simulink model "sschdlexPMSMDriveOptimizedMotor"  (R2026a)
settings: Solver=FixedStepDiscrete  StopTime=0.6  AbsTol=1e-3
PreLoadFcn:
  | % Control parameters
  | Ts = 1e-6;   % Fundamental sample time
  | fsw = 25e3;   % Switching frequency (Hz)
  | fc = fsw*10; % Control loop frequency (Hz)
  | Tsc = 1/fc;  % Control loop sample time
  | 
  | % PMSM parameters
  | PM = 0.03; % Permanent magnet flux linkage
  | Ld = 2e-4;  % d-axis inductance
  | Lq = 2e-4;  % q-axis inductance
  | L0 = 2e-4;  % 0-axis inductance
  | Rs = 0.013; % Stator resistance
  | N = 6; % Number of pole pairs
  | J = 0.2; % Moment of inertia
  | 
  | % Operating and derived limits
  | Imax = 100;  % Max stator current (peak value)
  | Tmax = 1.5*N*PM*Imax; % Max lectromagnetic torque
  | fnom = 100;  % Nominal frequency (Hz)
  | rpm_nom = 60*fnom/N;      % Nominal rotor speed (rpm)
  | omegam_nom = 2*pi*fnom/N; % Nominal mechanical rotor speed
  | Pmax = omegam_nom*Tmax;     % Maximum power
  | 
  | Gs = 4.4526;
  | s = 2.8994;
  | h = 2e-6;
PostLoadFcn:
  | SimscapePlant_SolverConfiguration_Gs = Simulink.Parameter;
  | SimscapePlant_SolverConfiguration_Gs.Value = 1;
  | SimscapePlant_SolverConfiguration_Gs.CoderInfo.StorageClass = 'ExportedGlobal';
  | SimscapePlant_SolverConfiguration_s = Simulink.Parameter;
  | SimscapePlant_SolverConfiguration_s.Value = 1;
  | SimscapePlant_SolverConfiguration_s.CoderInfo.StorageClass = 'ExportedGlobal';SimscapePlant_PermanentMagnetSynchronousMotor_NPP = Simulink.Parameter;
  | SimscapePlant_PermanentMagnetSynchronousMotor_NPP.Value = 6;
  | SimscapePlant_PermanentMagnetSynchronousMotor_NPP.CoderInfo.StorageClass = 'ExportedGlobal';SimscapePlant_PermanentMagnetSynchronousMotor_Lambda_pm = Simulink.Parameter;
  | SimscapePlant_PermanentMagnetSynchronousMotor_Lambda_pm.Value = 0.03;
  | SimscapePlant_PermanentMagnetSynchronousMotor_Lambda_pm.CoderInfo.StorageClass = 'ExportedGlobal';SimscapePlant_PermanentMagnetSynchronousMotor_Ld = Simulink.Parameter;
  | SimscapePlant_PermanentMagnetSynchronousMotor_Ld.Value = 0.0002;
  | SimscapePlant_PermanentMagnetSynchronousMotor_Ld.CoderInfo.StorageClass = 'ExportedGlobal';SimscapePlant_PermanentMagnetSynchronousMotor_Lq = Simulink.Parameter;
  | SimscapePlant_PermanentMagnetSynchronousMotor_Lq.Value = 0.0002;
  | SimscapePlant_PermanentMagnetSynchronousMotor_Lq.CoderInfo.StorageClass = 'ExportedGlobal';SimscapePlant_PermanentMagnetSynchronousMotor_Rs = Simulink.Parameter;
  | SimscapePlant_PermanentMagnetSynchronousMotor_Rs.Value = 0.013;
  | SimscapePlant_PermanentMagnetSynchronousMotor_Rs.CoderInfo.StorageClass = 'ExportedGlobal';
libraries: SimscapeFPGAHIL_lib x13, nesl_utility x7, fl_lib x6, ee_lib x3, eePmsmFieldOrientedControl x1, batteryecm_lib x1
Description:
  | Three-Phase PMSM Drive
settings Model: DataTypeOverride=Off  Creator=The MathWorks, Inc.  LastModifiedBy=The MathWorks, Inc.
settings SolverCC: MaxConsecutiveMinStep=2  ZeroCrossAlgorithm=Adaptive
settings DataIOCC: MaxDataPoints=690000  SignalLoggingName=logsout_ee_pmsm_drive
settings OptimizationCC: ConditionallyExecuteInputs=off  InheritOutputTypeSmallerThanSingle=on
settings DebuggingCC: AlgebraicLoopMsg=error  MaxConsecutiveZCsMsg=none  IgnoredZcDiagnostic=none  SingleTaskRateTransMsg=error  ParameterPrecisionLossMsg=none  PregeneratedLibrarySubsystemCodeDiagnostic=none
settings HardwareCC: ProdHWDeviceType=ASIC/FPGA->ASIC/FPGA  TargetBitPerLong=64.0  TargetBitPerPointer=64.0  TargetBitPerSizeT=64.0  TargetBitPerPtrDiffT=64.0  TargetLongLongMode=on  TargetIntDivRoundTo=Zero  TargetEndianess=LittleEndian  TargetWordSize=64.0  TargetHWDeviceType=Custom Processor->MATLAB Host Computer  ProdEqTarget=off
settings SimscapeCC: SimscapeNominalValues="[{\"value\":\"1\",\"unit\":\"A\"},{\"value\":\"1\",\"unit\":\"bar\"},{\"value\":\"1\",\"unit\":\"cm^2\"},{\"value\":\"1\",\"unit\":\"cm^3/s\"},{\"value\":\"1\",\"unit\":\"kJ/kg\"},{\"value\":\"1\",\"unit\":\"kW\"},{\"value\":\"1\",\"unit\":\"l\"},{\"value\":\"1\",\"unit\":\"N\"},{\"value\":\"1\",\"unit\":\"N*m\"},{\"value\":\"1\",\"unit\":\"V\"}]"  SimscapeLogSimulationStatistics=on  SimscapeLogName=simlog_ee_pmsm_drive  SimscapeLogDataHistory=690000.0

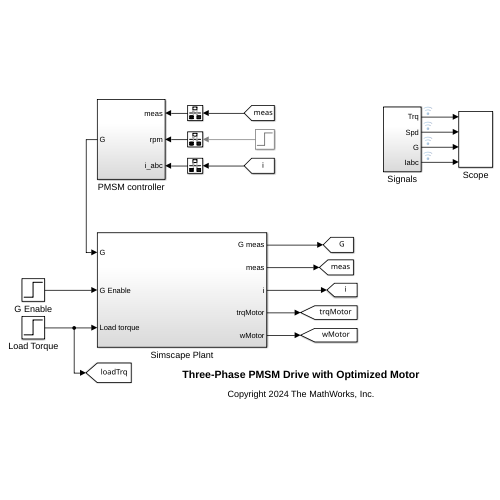
[thumbnail: Simulink's stored preview of the top-level diagram]
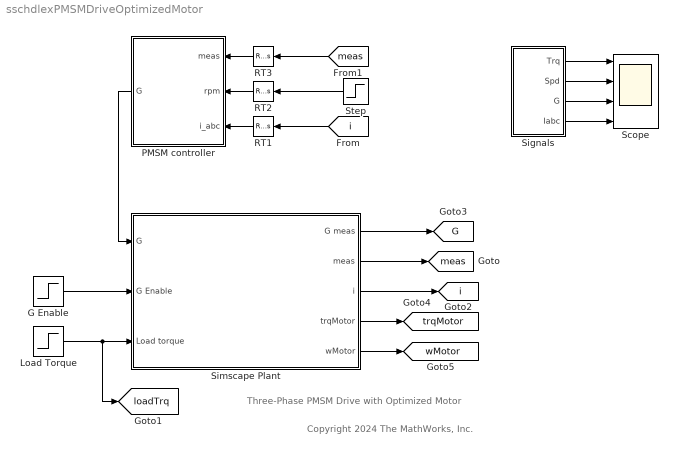
== system sschdlexPMSMDriveOptimizedMotor ==
  note: Three-Phase PMSM Drive with Optimized Motor
  note: Copyright 2024 The MathWorks, Inc.
  G Enable : Step  Time=1e-4  SampleTime=Ts
  Load Torque : Step  Time=0.1  FinalValue=5  SampleTime=Ts
  PMSM controller : Subsystem
  RT1 : RateTransition  OutPortSampleTime=Tsc
  RT2 : RateTransition  OutPortSampleTime=Tsc
  RT3 : RateTransition  OutPortSampleTime=Tsc
  Scope : Scope  NumInputPorts=4
      settings: Title=Demanded and achieved torques  ActiveDisplayYMinimum=-0.625  ActiveDisplayYMaximum=5.625
  "Signals " : Subsystem
  Simscape Plant : Subsystem
  Step : Step  Time=0.1  FinalValue=500  SampleTime=0
  tag scope: G=global, i=global, loadTrq=global, meas=global, trqMotor=global, wMotor=global
  wires:
  Step/1 -> RT2/1
  RT3/1 -> PMSM controller/1(meas)
  RT2/1 -> PMSM controller/2(rpm)
  RT1/1 -> PMSM controller/3(i_abc)
  "Signals "/2(Spd) -> Scope/2
  "Signals "/4(Iabc) -> Scope/4
  "Signals "/3(G) -> Scope/3
  "Signals "/1(Trq) -> Scope/1
  [i] -> RT1/1
  [meas] -> RT3/1
  PMSM controller/1(G) -> Simscape Plant/1(G)
  G Enable/1 -> Simscape Plant/2(G Enable)
  Load Torque/1 -> [loadTrq], Simscape Plant/3(Load torque)
  Simscape Plant/2(meas) -> [meas]
  Simscape Plant/3(i) -> [i]
  Simscape Plant/1(G meas) -> [G]
  Simscape Plant/4(trqMotor) -> [trqMotor]
  Simscape Plant/5(wMotor) -> [wMotor]

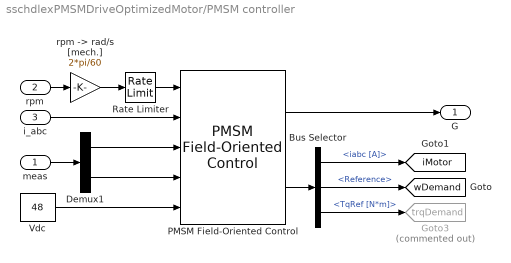
== system sschdlexPMSMDriveOptimizedMotor/PMSM controller ==
  meas : Inport
  rpm : Inport  Port=2
  i_abc : Inport  Port=3
  Bus Selector : BusSelector  OutputSignals=iabc [A],Reference,TqRef [N*m]
  Demux1 : Demux  Outputs=2
  Goto3 : Goto  Commented=on  GotoTag=trqDemand  TagVisibility=global
  PMSM Field-Oriented Control : eePmsmFieldOrientedControl/PMSM Field-Oriented Control  winding_type=Wye-wound  CtrlMode=Velocity control  Vnom=48  Pmax=Pmax  Tmax=Tmax*1.5  p=N  Vdc_on=10  Ts=Ts  Tsc=Tsc  CtrlType=PI control  Kp_w=60  Ki_w=300*2  Kv_w=1  Kaw_w=1000  RefType=Zero d-axis control  rpmVec=[0, 3000]  TqVec=[-100, 0, 100]  VdcVec=[300, 350]  PWMMode=SPWM: sinusoidal PWM  ModFactor=1  idMatrix=zeros(2,3,2)  iqMatrix=zeros(2,3,2)  psim=PM  Ld=0.00024  Lq=0.00029  Rs=0.01  AxisAlignment=Q-axis  Kp_id=0.1  Ki_id=10  Kaw_id=1000  Kp_iq=0.1  Ki_iq=10  Kaw_iq=1000  AxisPrio=Q-axis  ActZC=off  ActFF=on  ParamTypeFF=Constant parameters  LdFF=Ld  LqFF=Lq  psimFF=PM  idVect=[-200, 0, 200]  iqVect=[-200, 0, 200]  LdMatrix=0.0002 * ones(3, 3)  LqMatrix=0.0002 * ones(3, 3)  psimMatrix=0.04 * ones(3, 3)  CPWMMode=SPWM: sinusoidal PWM  fsw=fsw
  Rate Limiter : RateLimiter  RisingSlewLimit=Tmax/J  FallingSlewLimit=-Tmax/J  SampleTimeMode=inherited
  Vdc : Constant  Value=48  SampleTime=Tsc
  "rpm -> rad/s [mech.]" : Gain  Gain=2*pi/60
  G : Outport  VectorParamsAs1DForOutWhenUnconnected=off
  tag scope: iMotor=global, wDemand=global
  wires:
  PMSM Field-Oriented Control/1 -> G/1
  Vdc/1 -> PMSM Field-Oriented Control/5
  PMSM Field-Oriented Control/2 -> Bus Selector/1
  i_abc/1 -> PMSM Field-Oriented Control/2
  meas/1 -> Demux1/1
  Demux1/1 -> PMSM Field-Oriented Control/3
  Demux1/2 -> PMSM Field-Oriented Control/4
  Bus Selector/1 -> [iMotor]  "<iabc [A]>"
  Bus Selector/2 -> [wDemand]  "<Reference>"
  Bus Selector/3 -> Goto3/1  "<TqRef [N*m]>"
  rpm/1 -> "rpm -> rad/s [mech.]"/1
  Rate Limiter/1 -> PMSM Field-Oriented Control/1
  "rpm -> rad/s [mech.]"/1 -> Rate Limiter/1

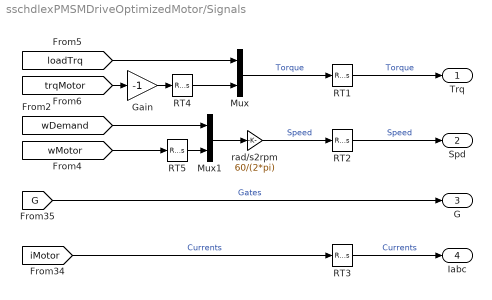
== system sschdlexPMSMDriveOptimizedMotor/Signals  ==
  Gain : Gain  Gain=-1
  Mux : Mux  Inputs=2
  Mux1 : Mux  Inputs=2
  RT{1..4} (4 alike) : RateTransition  OutPortSampleTime=Ts
  RT5 : RateTransition  OutPortSampleTime=Tsc
  rad/s2rpm : Gain  Gain=60/(2*pi)
  Trq : Outport  VectorParamsAs1DForOutWhenUnconnected=off
  Spd : Outport  Port=2  VectorParamsAs1DForOutWhenUnconnected=off
  G : Outport  Port=3  VectorParamsAs1DForOutWhenUnconnected=off
  Iabc : Outport  Port=4  VectorParamsAs1DForOutWhenUnconnected=off
  wires:
  [loadTrq] -> Mux/1
  [G] -> G/1  "Gates"
  Mux1/1 -> rad/s2rpm/1
  Mux/1 -> RT1/1  "Torque"
  [iMotor] -> RT3/1  "Currents"
  [wDemand] -> Mux1/1
  rad/s2rpm/1 -> RT2/1  "Speed"
  [trqMotor] -> Gain/1
  [wMotor] -> RT5/1
  RT1/1 -> Trq/1  "Torque"
  RT2/1 -> Spd/1  "Speed"
  RT3/1 -> Iabc/1  "Currents"
  RT4/1 -> Mux/2
  RT5/1 -> Mux1/2
  Gain/1 -> RT4/1

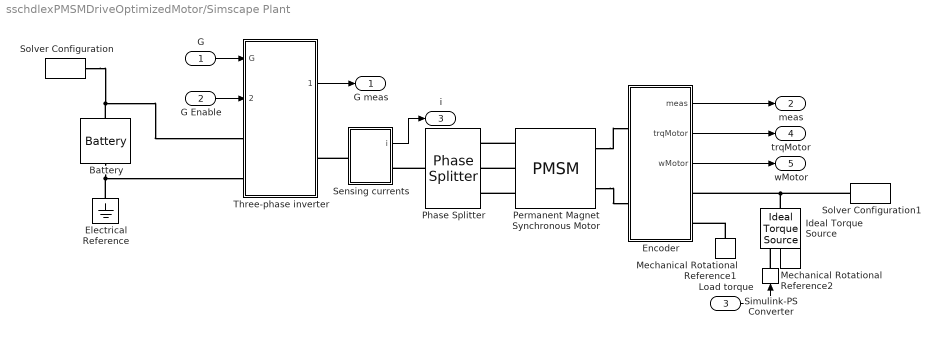
== system sschdlexPMSMDriveOptimizedMotor/Simscape Plant ==
  G : Inport
  G Enable : Inport  Port=2
  Load torque : Inport  Port=3
  Battery : batteryecm_lib/Battery  Vnom=48 V  prm_dir=1  R1_dis=2 Ohm  R1_ch=2 Ohm  R1=0.001 Ohm  prm_AH=1  AH=14000 hr*A  V1=470 V  AH1=5000 hr*A  prm_R2=1  R2=inf Ohm  Tmeas=298.15 K  charge_measurement_port=simscape.enum.battery.enable.no  prm_dyn=1  Rp1=0.005 Ohm  tau1=30 s  Rp2=0.005 Ohm  tau2=30 s  Rp3=0.005 Ohm  tau3=30 s  Rp4=0.005 Ohm  tau4=30 s  Rp5=0.005 Ohm  tau5=30 s  prm_fade=1  N_fade=100  AH_fade=45 hr*A  R1_fade=2.02 Ohm  R1_ch_fade=2.02 Ohm  V1_fade=10.35 V  prm_age=1  prm_age_OCV=1  OCV_age=0.9  SOC_age=60  Tmeas_age=298.15 K  delta_time_age_vec=[0] d  temperature_age_vec=[273] K  OCV_scaling_age=2.2134e6  OCV_offset_age=1.632e6  temp_exp_age=0.515833569 V  t_exp_age=0.75  Vnom_T2=12 V  R1_T2=2.2 Ohm  R1_T2_dis=2.2 Ohm  R1_T2_ch=2.2 Ohm  V1_T2=11.4 V  R2_T2=2200 Ohm  Rp1_T2=0.005 Ohm  tau1_T2=30 s  Rp2_T2=0.005 Ohm  tau2_T2=30 s  Rp3_T2=0.005 Ohm  tau3_T2=30 s  Rp4_T2=0.005 Ohm  tau4_T2=30 s  Rp5_T2=0.005 Ohm  tau5_T2=30 s  Tmeas2=273.15 K  thermal_port=simscape.enum.thermaleffects.omit  thermal_mass=30000 J/K  i_specify=off  i_priority=None  i=0 A  i_nominal_specify=off  i_nominal_value=1  i_nominal_unit=A  v_specify=off  v_priority=None  v=0 V  v_nominal_specify=off  v_nominal_value=1  v_nominal_unit=V  charge_specify=on  charge_priority=High  charge=7000 hr*A  charge_nominal_specify=off  charge_nominal_value=1  charge_nominal_unit=A*hr  num_cycles_specify=off  num_cycles_priority=High  num_cycles=0  num_cycles_nominal_specify=off  num_cycles_nominal_value=1  num_cycles_nominal_unit=1  temperature_specify=off  temperature_priority=High  temperature=298.15 K  temperature_nominal_specify=off  temperature_nominal_value=1  temperature_nominal_unit=K
  Electrical Reference : fl_lib/Electrical/Electrical Elements/Electrical Reference
  Encoder : Subsystem
  Ideal Torque Source : fl_lib/Mechanical/Mechanical Sources/Ideal Torque Source
  Mechanical Rotational Reference1 : fl_lib/Mechanical/Rotational Elements/Mechanical Rotational Reference
  Mechanical Rotational Reference2 : fl_lib/Mechanical/Rotational Elements/Mechanical Rotational Reference
  Permanent Magnet Synchronous Motor : SimscapeFPGAHIL_lib/PMSM Motor/PMSM  NPP=SimscapePlant_PermanentMagnetSynchronousMotor_NPP  Lambda_pm=SimscapePlant_PermanentMagnetSynchronousMotor_Lambda_pm  Ld=SimscapePlant_PermanentMagnetSynchronousMotor_Ld  Lq=SimscapePlant_PermanentMagnetSynchronousMotor_Lq  Rs=SimscapePlant_PermanentMagnetSynchronousMotor_Rs  J=0.2  winding=Wye  Load_type=Torque-driven  Ts=Ts  torque_initial=0  i_d_initial=0  i_q_initial=0  angular_position_initial=0  angular_velocity_initial=0
  Phase Splitter : ee_lib/Connectors & References/Phase Splitter
  Sensing currents : Subsystem
      mask Display: disp('i')
  Simulink-PS Converter : nesl_utility/Simulink-PS Converter  PhysicalDomain=network_engine_domain  SubClassName=ps_input  LeftPortType=input  RightPortType=output  PseudoPeriodic=off  Frequencies=[]  NoiseDistribution=none  NoiseParameters=[]  Unit=1  AffineConversion=off  FilteringAndDerivatives=provide  SimscapeFilterOrder=1  InputFilterTimeConstant=0.001  UdotUserProvided=0
  Solver Configuration : nesl_utility/Solver Configuration  PhysicalDomain=network_engine_domain  SubClassName=solver  LeftPortType=input  RightPortType=generic  Tones=[]  Harmonics=[]  SimulateNoise=off  Profile=off  UseLocalSampling=off  EnableSwitchedLinearOptims=on  FrequencyDomain=off  UseCCode=off  RelTol=0.001  AbsTol=1e-06  MinStep=1e-09  ToWorkspace=off  RevertToSquareIcSolve=off  NumHomotopyIterations=100  PhasorMode=off  PhasorModeNumHarmonics=1  ConsistencySolver=NEWTON_FTOL  CanonicalOrdering=UNORDERED  OptimizeIntermediates=UNOPTIMIZED  IndexReductionMethod=DerivativeReplacement  DoDC=off  ResidualTolerance=1e-9  ConsistencyTolSource=GLOBAL  ConsistencyAbsTol=0.001  ConsistencyRelTol=0.001  ConsistencyTolFactor=0.001  UseLocalSolver=on  LocalSolverChoice=NE_BACKWARD_EULER_ADVANCER  ResolveIndetEquations=on  FunctionEvalNumThread=1  LocalSolverSampleTime=Ts  DoFixedCost=on  MaxNonlinIter=4  MaxModeIter=2  ComputeImpulses=off  ImpulseIterations=2  LinearAlgebra=auto  LinearAlgebraNumThread=0  EquationFormulation=NE_TIME_EF  DelaysMemoryBudget=1024  AutomaticFiltering=on  FilteringTimeConstant=0.001  PartitionStorageMethod=AS_NEEDED  PartitionMemoryBudget=1024  PartitionMethod=FAST  MultibodyUseLocalSolver=off  MultibodyLocalSolverChoice=ODE1  MultibodyLocalSolverSampleTime=0.001
  Solver Configuration1 : nesl_utility/Solver Configuration  PhysicalDomain=network_engine_domain  SubClassName=solver  LeftPortType=input  RightPortType=generic  Tones=[]  Harmonics=[]  SimulateNoise=off  Profile=off  UseLocalSampling=off  EnableSwitchedLinearOptims=on  FrequencyDomain=off  UseCCode=off  RelTol=0.001  AbsTol=1e-06  MinStep=1e-09  ToWorkspace=off  RevertToSquareIcSolve=off  NumHomotopyIterations=100  PhasorMode=off  PhasorModeNumHarmonics=1  ConsistencySolver=NEWTON_FTOL  CanonicalOrdering=UNORDERED  OptimizeIntermediates=UNOPTIMIZED  IndexReductionMethod=DerivativeReplacement  DoDC=off  ResidualTolerance=1e-9  ConsistencyTolSource=GLOBAL  ConsistencyAbsTol=0.001  ConsistencyRelTol=0.001  ConsistencyTolFactor=0.001  UseLocalSolver=on  LocalSolverChoice=NE_BACKWARD_EULER_ADVANCER  ResolveIndetEquations=on  FunctionEvalNumThread=1  LocalSolverSampleTime=Ts  DoFixedCost=on  MaxNonlinIter=4  MaxModeIter=2  ComputeImpulses=off  ImpulseIterations=2  LinearAlgebra=auto  LinearAlgebraNumThread=0  EquationFormulation=NE_TIME_EF  DelaysMemoryBudget=1024  AutomaticFiltering=on  FilteringTimeConstant=0.001  PartitionStorageMethod=AS_NEEDED  PartitionMemoryBudget=1024  PartitionMethod=FAST  MultibodyUseLocalSolver=off  MultibodyLocalSolverChoice=ODE1  MultibodyLocalSolverSampleTime=0.001
  Three-phase inverter : Subsystem
  G meas : Outport
  meas : Outport  Port=2
  i : Outport  Port=3
  trqMotor : Outport  Port=4
  wMotor : Outport  Port=5
  wires:
  G Enable/1 -> Three-phase inverter/2(G Enable)
  Load torque/1 -> Simulink-PS Converter/1
  Encoder/1(meas) -> meas/1
  G/1 -> Three-phase inverter/1(G)
  Sensing currents/1(i) -> i/1
  Three-phase inverter/1(G meas) -> G meas/1
  Encoder/3(wMotor) -> wMotor/1
  Encoder/2(trqMotor) -> trqMotor/1
  connections:
  Solver Configuration/RConn1 -- Three-phase inverter/LConn1 -- Battery/LConn1
  Mechanical Rotational Reference1/LConn1 -- Encoder/RConn2
  Sensing currents/LConn1 -- Three-phase inverter/RConn1
  Ideal Torque Source/RConn2 -- Mechanical Rotational Reference2/LConn1
  Ideal Torque Source/LConn1 -- Encoder/RConn1 -- Solver Configuration1/RConn1
  Simulink-PS Converter/RConn1 -- Ideal Torque Source/RConn1
  Electrical Reference/LConn1 -- Battery/RConn1 -- Three-phase inverter/LConn2
  Phase Splitter/LConn1 -- Sensing currents/RConn1
  Permanent Magnet Synchronous Motor/RConn2 -- Encoder/LConn2
  Permanent Magnet Synchronous Motor/LConn2 -- Phase Splitter/RConn2
  Permanent Magnet Synchronous Motor/RConn1 -- Encoder/LConn1
  Permanent Magnet Synchronous Motor/LConn1 -- Phase Splitter/RConn1
  Permanent Magnet Synchronous Motor/LConn3 -- Phase Splitter/RConn3

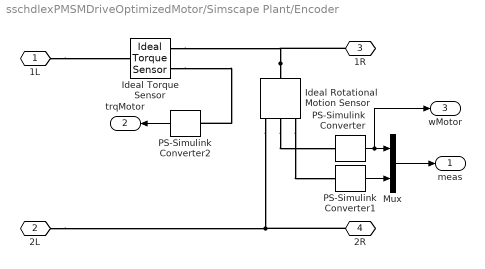
== system sschdlexPMSMDriveOptimizedMotor/Simscape Plant/Encoder ==
  Ideal Rotational Motion Sensor : fl_lib/Mechanical/Mechanical Sensors/Ideal Rotational Motion Sensor  reference=foundation.enum.MeasurementReference.difference  acceleration_port=false  velocity_port=true  position_port=true  wrap_angle=simscape.enum.onoff.off  offset=0 deg
  Ideal Torque Sensor : fl_lib/Mechanical/Mechanical Sensors/Ideal Torque Sensor
  Mux : Mux  Inputs=2
  PS-Simulink Converter : nesl_utility/PS-Simulink Converter  PhysicalDomain=network_engine_domain  SubClassName=ps_output  LeftPortType=input  RightPortType=output  PseudoPeriodic=off  Frequencies=[]  VectorFormat=1-D array  Unit=rad/s  AffineConversion=off
  PS-Simulink Converter1 : nesl_utility/PS-Simulink Converter  PhysicalDomain=network_engine_domain  SubClassName=ps_output  LeftPortType=input  RightPortType=output  PseudoPeriodic=off  Frequencies=[]  VectorFormat=1-D array  Unit=rad  AffineConversion=off
  PS-Simulink Converter2 : nesl_utility/PS-Simulink Converter  PhysicalDomain=network_engine_domain  SubClassName=ps_output  LeftPortType=input  RightPortType=output  PseudoPeriodic=off  Frequencies=[]  VectorFormat=1-D array  Unit=N*m  AffineConversion=off
  1L : PMIOPort  Side=Left
  2L : PMIOPort  Port=2  Side=Left
  1R : PMIOPort  Port=3  Side=Right
  2R : PMIOPort  Port=4  Side=Right
  meas : Outport  VectorParamsAs1DForOutWhenUnconnected=off
  trqMotor : Outport  Port=2
  wMotor : Outport  Port=3
  wires:
  PS-Simulink Converter2/1 -> trqMotor/1
  Mux/1 -> meas/1
  PS-Simulink Converter1/1 -> Mux/2
  PS-Simulink Converter/1 -> wMotor/1, Mux/1
  connections:
  Ideal Torque Sensor/RConn2 -- PS-Simulink Converter2/LConn1
  1L/RConn1 -- Ideal Torque Sensor/LConn1
  2R/RConn1 -- 2L/RConn1 -- Ideal Rotational Motion Sensor/RConn1
  Ideal Rotational Motion Sensor/LConn1 -- 1R/RConn1 -- Ideal Torque Sensor/RConn1
  Ideal Rotational Motion Sensor/RConn2 -- PS-Simulink Converter/LConn1
  Ideal Rotational Motion Sensor/RConn3 -- PS-Simulink Converter1/LConn1

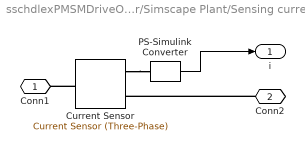
== system sschdlexPMSMDriveOptimizedMotor/Simscape Plant/Sensing currents ==
  Current Sensor : ee_lib/Sensors & Transducers/Current Sensor (Three-Phase)  port_option=ee.enum.threePhasePort.composite
  PS-Simulink Converter : nesl_utility/PS-Simulink Converter  PhysicalDomain=network_engine_domain  SubClassName=ps_output  LeftPortType=input  RightPortType=output  PseudoPeriodic=off  Frequencies=[]  VectorFormat=1-D array  Unit=A  AffineConversion=off
  Conn1 : PMIOPort  Side=Left
  Conn2 : PMIOPort  Port=2  Side=Right
  i : Outport
  wires:
  PS-Simulink Converter/1 -> i/1
  connections:
  Current Sensor/RConn1 -- PS-Simulink Converter/LConn1
  Conn2/RConn1 -- Current Sensor/RConn2
  Current Sensor/LConn1 -- Conn1/RConn1

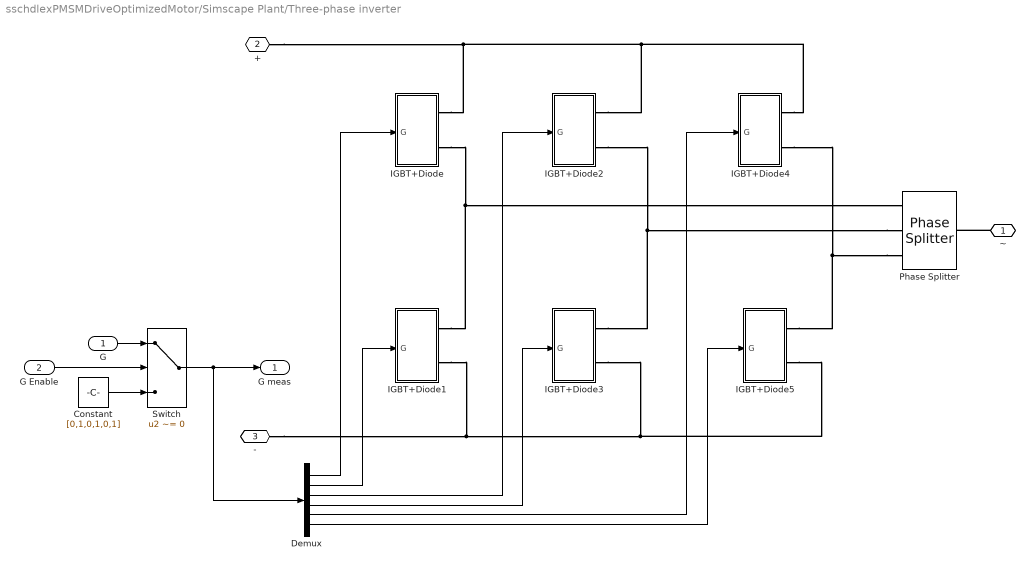
== system sschdlexPMSMDriveOptimizedMotor/Simscape Plant/Three-phase inverter ==
  G : Inport
  G Enable : Inport  Port=2
  Constant : Constant  Value=[0,1,0,1,0,1]  SampleTime=-1
  Demux : Demux  Outputs=6
  IGBT+Diode : Subsystem
  IGBT+Diode1 : Subsystem
  IGBT+Diode2 : Subsystem
  IGBT+Diode3 : Subsystem
  IGBT+Diode4 : Subsystem
  IGBT+Diode5 : Subsystem
  Phase Splitter : ee_lib/Connectors & References/Phase Splitter
  Switch : Switch  Criteria=u2 ~= 0  SaturateOnIntegerOverflow=off  InputSameDT=off
  ~ : PMIOPort  Tag=PMCPort  Side=Right
  + : PMIOPort  Tag=PMCPort  Port=2  Side=Left
  - : PMIOPort  Tag=PMCPort  Port=3  Side=Left
  G meas : Outport
  wires:
  Switch/1 -> G meas/1, Demux/1
  Demux/2 -> IGBT+Diode1/1(G)
  Demux/3 -> IGBT+Diode2/1(G)
  Demux/4 -> IGBT+Diode3/1(G)
  Demux/5 -> IGBT+Diode4/1(G)
  Demux/6 -> IGBT+Diode5/1(G)
  Demux/1 -> IGBT+Diode/1(G)
  G/1 -> Switch/1
  Constant/1 -> Switch/3
  G Enable/1 -> Switch/2
  connections:
  Phase Splitter/RConn3 -- IGBT+Diode5/RConn1 -- IGBT+Diode4/RConn2
  ~/RConn1 -- Phase Splitter/LConn1
  IGBT+Diode/RConn2 -- IGBT+Diode1/RConn1 -- Phase Splitter/RConn1
  +/RConn1 -- IGBT+Diode4/RConn1 -- IGBT+Diode2/RConn1 -- IGBT+Diode/RConn1
  Phase Splitter/RConn2 -- IGBT+Diode3/RConn1 -- IGBT+Diode2/RConn2
  IGBT+Diode1/RConn2 -- -/RConn1 -- IGBT+Diode3/RConn2 -- IGBT+Diode5/RConn2

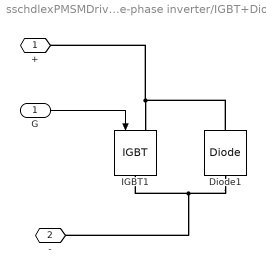
== system sschdlexPMSMDriveOptimizedMotor/Simscape Plant/Three-phase inverter/IGBT+Diode ==
  G : Inport
  Diode1 : SimscapeFPGAHIL_lib/Dynamic Switch Models/Diode  Vf=0.8  Gs=Gs  s=s
  IGBT1 : SimscapeFPGAHIL_lib/Dynamic Switch Models/IGBT  Vf=0.8  Vth=0.5  Gs=Gs  s=s
  + : PMIOPort  Side=Right
  - : PMIOPort  Port=2  Side=Right
  wires:
  G/1 -> IGBT1/1
  connections:
  -/RConn1 -- Diode1/LConn1 -- IGBT1/RConn1
  +/RConn1 -- Diode1/RConn1 -- IGBT1/LConn1

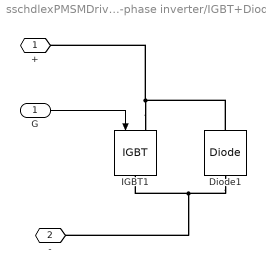
== system sschdlexPMSMDriveOptimizedMotor/Simscape Plant/Three-phase inverter/IGBT+Diode1 ==
  G : Inport
  Diode1 : SimscapeFPGAHIL_lib/Dynamic Switch Models/Diode  Vf=0.8  Gs=Gs  s=s
  IGBT1 : SimscapeFPGAHIL_lib/Dynamic Switch Models/IGBT  Vf=0.8  Vth=0.5  Gs=Gs  s=s
  + : PMIOPort  Side=Right
  - : PMIOPort  Port=2  Side=Right
  wires:
  G/1 -> IGBT1/1
  connections:
  IGBT1/LConn1 -- +/RConn1 -- Diode1/RConn1
  IGBT1/RConn1 -- Diode1/LConn1 -- -/RConn1

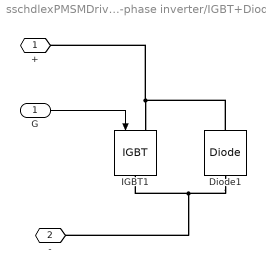
== system sschdlexPMSMDriveOptimizedMotor/Simscape Plant/Three-phase inverter/IGBT+Diode2 ==
  G : Inport
  Diode1 : SimscapeFPGAHIL_lib/Dynamic Switch Models/Diode  Vf=0.8  Gs=Gs  s=s
  IGBT1 : SimscapeFPGAHIL_lib/Dynamic Switch Models/IGBT  Vf=0.8  Vth=0.5  Gs=Gs  s=s
  + : PMIOPort  Side=Right
  - : PMIOPort  Port=2  Side=Right
  wires:
  G/1 -> IGBT1/1
  connections:
  -/RConn1 -- Diode1/LConn1 -- IGBT1/RConn1
  Diode1/RConn1 -- +/RConn1 -- IGBT1/LConn1

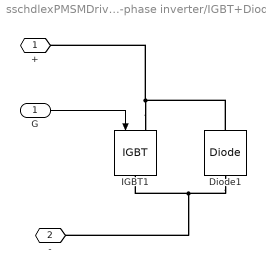
== system sschdlexPMSMDriveOptimizedMotor/Simscape Plant/Three-phase inverter/IGBT+Diode3 ==
  G : Inport
  Diode1 : SimscapeFPGAHIL_lib/Dynamic Switch Models/Diode  Vf=0.8  Gs=Gs  s=s
  IGBT1 : SimscapeFPGAHIL_lib/Dynamic Switch Models/IGBT  Vf=0.8  Vth=0.5  Gs=Gs  s=s
  + : PMIOPort  Side=Right
  - : PMIOPort  Port=2  Side=Right
  wires:
  G/1 -> IGBT1/1
  connections:
  IGBT1/LConn1 -- +/RConn1 -- Diode1/RConn1
  IGBT1/RConn1 -- Diode1/LConn1 -- -/RConn1

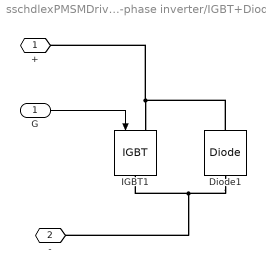
== system sschdlexPMSMDriveOptimizedMotor/Simscape Plant/Three-phase inverter/IGBT+Diode4 ==
  G : Inport
  Diode1 : SimscapeFPGAHIL_lib/Dynamic Switch Models/Diode  Vf=0.8  Gs=Gs  s=s
  IGBT1 : SimscapeFPGAHIL_lib/Dynamic Switch Models/IGBT  Vf=0.8  Vth=0.5  Gs=Gs  s=s
  + : PMIOPort  Side=Right
  - : PMIOPort  Port=2  Side=Right
  wires:
  G/1 -> IGBT1/1
  connections:
  -/RConn1 -- Diode1/LConn1 -- IGBT1/RConn1
  Diode1/RConn1 -- +/RConn1 -- IGBT1/LConn1

== system sschdlexPMSMDriveOptimizedMotor/Simscape Plant/Three-phase inverter/IGBT+Diode5 ==
  G : Inport
  Diode1 : SimscapeFPGAHIL_lib/Dynamic Switch Models/Diode  Vf=0.8  Gs=Gs  s=s
  IGBT1 : SimscapeFPGAHIL_lib/Dynamic Switch Models/IGBT  Vf=0.8  Vth=0.5  Gs=Gs  s=s
  + : PMIOPort  Side=Right
  - : PMIOPort  Port=2  Side=Right
  wires:
  G/1 -> IGBT1/1
  connections:
  IGBT1/LConn1 -- +/RConn1 -- Diode1/RConn1
  IGBT1/RConn1 -- Diode1/LConn1 -- -/RConn1
